simulink model "tsc_control_red"  (R2024a)
settings: Solver=ode15s  StartTime=0.0  StopTime=tm_final  MaxStep=tm_h  RelTol=1e-9  AbsTol=1e-11
model workspace (MAT data in the model file):
  tm_C1 = 1.87501784269e-05
  tm_C2 = 3.75003568539e-05
  tm_Cp = 2.89288467158e-06
  tm_L1 = 0.26018031666
  tm_L2 = 0.13009015833
  tm_Lg = 0.0008
  tm_R1 = 1.15690788571
  tm_R2 = 0.578453942857
  tm_Rb1 = 84640
  tm_Rb2 = 42320
  tm_Rg = 0.4
  tm_Rp = 2.20064
  tm_a1 = 1
  tm_a2 = 0.03
  tm_a3 = 0.03
  tm_carga = [0 1e-05 2e-05 3e-05 4e-05 5e-05 6e-05 7e-05 8e-05 9e-05 0.0001 0.00011 ... (160002 elements, 80001x2)]
  tm_final = 0.8
  tm_h = 2.5e-05
  tm_iG0 = 2.93102214056
  tm_lambda = 229.793279031
  tm_omega = 314.159265359
  tm_vC10 = 0
  tm_vC20 = 0
  tm_vCp0 = 342.613901809
  tsc_cfg.p.L_H = [0.26018031666 0.13009015833]
  tsc_cfg.p.C_F = [1.87501784269e-05 3.75003568539e-05]
  tsc_cfg.p.R_ohm = [1.15690788571 0.578453942857]
  tsc_cfg.p.Rb_ohm = [84640 42320]
  tsc_cfg.p.Cp_F = 2.89288467158e-06
  tsc_cfg.p.Rp_ohm = 2.20064
  tsc_cfg.p.omega = 314.159265359
  tsc_cfg.p.T = 0.02
  tsc_cfg.p.lambda = 229.793279031
  tsc_cfg.p.k = 42.32
  tsc_cfg.p.coefTension = [1 0.03 0.03]
  tsc_cfg.p.limiteDiDt_A_s = 2500
  tsc_cfg.p.limiteDiDtPlan_A_s = 2475
  tsc_cfg.p.margenDiDt = 0.01
  tsc_cfg.p.permanenciaMin_s = 0.06
  tsc_cfg.p.histeresis_A2 = 0.025
  tsc_cfg.p.pasoMuestreo_s = 0.00031746031746
  tsc_cfg.p.ruidoSigma_A = 0
  tsc_cfg.p.PNominal_W = 1000
  tsc_cfg.p.opciones.CasoTension = "moderada"
  tsc_cfg.p.opciones.Modo = "ga"
  tsc_cfg.p.opciones.BitsFijos = [1 0]
  tsc_cfg.p.opciones.PNominal_W = 1000
  tsc_cfg.p.opciones.Duracion_s = 0.8
  tsc_cfg.p.opciones.PasoMaximo_s = 2.5e-05
  tsc_cfg.p.opciones.VCInicial_V = [0 0]
  tsc_cfg.p.opciones.MaxDiDt_A_s = 2500
  tsc_cfg.p.opciones.Permanencia_s = 0.06
  tsc_cfg.p.opciones.Histeresis_A2 = 0.025
  tsc_cfg.p.opciones.MargenDiDt = 0.01
  tsc_cfg.p.opciones.EscalaCarga = [0.45 1.35 0.55 1.15]
  tsc_cfg.p.opciones.InstantesCarga_s = [0 0.2 0.4 0.6]
  tsc_cfg.p.opciones.Transicion_s = 0.06
  tsc_cfg.p.uReferencia = [344.475378053; 342.234056862; 335.572294082; 324.672808973; 309.827507389; 291.419626131; 269.900805928; 245.76494729; 219.520945261; 191.666460359; 162.664759213; 132.926361149; 102.796783137; 72.5511245888; 42.3956243918; 12.4757090319; -17.1105133821; -46.2948235646; -75.0193622969; -103.216997622; -130.793561892; -157.613734298; -183.491988067; -208.189539599; -231.417673404; -252.847222623; -272.123413738; -288.884787089; -302.784526411; -313.512304625; -320.814699368; -324.512354836; -324.512354836; -320.814699368; -313.512304625; -302.784526411; -288.884787089; -272.123413738; -252.847222623; -231.417673404; -208.189539599; -183.491988067; -157.613734298; -130.793561892; -103.216997622; -75.0193622969; -46.2948235646; -17.1105133821; 12.4757090319; 42.3956243918; 72.5511245888; 102.796783137; 132.926361149; 162.664759213; 191.666460359; 219.520945261; 245.76494729; 269.900805928; 291.419626131; 309.827507389; 324.672808973; 335.572294082; 342.234056862]
  tsc_cfg.p.iCargaReferencia = [6.51182189137; 7.16575638416; 7.73235116479; 8.21110783281; 8.60326005793; 8.91131348924; 9.13853778462; 9.2884553265; 9.3643709259; 9.36898275933; 9.30410728819; 9.17054063334; 8.96806671553; 8.69560948452; 8.35151387567; 7.9339288523; 7.44125698892; 6.87262928743; 6.22836178092; 5.51035213356; 4.72237972346; 3.87028111377; 2.9619836181; 2.00739188717; 1.01813500096; 0.00719333849221; -1.01156551506; -2.02390524428; -3.01575305312; -3.97370466865; -4.88546429102; -5.74018819674; -6.52870990668; -7.24363587413; -7.87931251943; -8.43167705693; -8.89801487251; -9.27665428601; -9.56663464748; -9.76738541319; -9.87845198541; -9.89929885692; -9.8292124672; -9.66731590084; -9.41269608903; -9.0646325672; -8.62290617078; -8.08815730582; -7.46225743332; -6.74865473042; -5.95265581387; -5.08160988616; -4.14496932337; -3.15421090963; -2.12261374764; -1.06490229599; 0.00322510035915; 1.06565147543; 2.10644175202; 3.11044532539; 4.06385658961; 4.95469208973; 5.77314935733]
  tsc_cfg.p.cpReferencia = [0.000821056838438 -0.0399433156679 -0.0796021803624 -0.11709608866 -0.151499211358 -0.182073153192 -0.208305554993 -0.229930479172 -0.246929145209 -0.259511271415 -0.268078939042 -0.273176379618 ... (126 elements, 63x2)]
  tsc_cfg.p.x0 = [0; 0; 0; 0; 0; 0]
  tsc_cfg.p.bits = [0  0; 0  1; 1  0; 1  1]
  tsc_cfg.D63 = [0 -10.0309181665 5.02170145378 -3.3547530699 2.52339001873 -2.02628170292 1.69632306201 -1.46190220008 1.28721732655 -1.15238243548 1.04546960893 -0.958891913625 ... (3969 elements, 63x63)]
  tsc_cfg.Modo = "ga"
  tsc_cfg.BitsFijos = [1 0]
  tsc_cfg.TsSupervision = 0.00031746031746
  tsc_cfg.Duracion_s = 0.8
  tsc_cfg.PasoMaximo_s = 2.5e-05
  tsc_cfg.VCInicial_V = [0 0]
  tsc_cfg.CasoTension = "moderada"
  tsc_cfg.opciones.CasoTension = "moderada"
  tsc_cfg.opciones.Modo = "ga"
  tsc_cfg.opciones.BitsFijos = [1 0]
  tsc_cfg.opciones.PNominal_W = 1000
  tsc_cfg.opciones.Duracion_s = 0.8
  tsc_cfg.opciones.PasoMaximo_s = 2.5e-05
  tsc_cfg.opciones.VCInicial_V = [0 0]
  tsc_cfg.opciones.MaxDiDt_A_s = 2500
  tsc_cfg.opciones.Permanencia_s = 0.06
  tsc_cfg.opciones.Histeresis_A2 = 0.025
  tsc_cfg.opciones.MargenDiDt = 0.01
  tsc_cfg.opciones.EscalaCarga = [0.45 1.35 0.55 1.15]
  tsc_cfg.opciones.InstantesCarga_s = [0 0.2 0.4 0.6]
  tsc_cfg.opciones.Transicion_s = 0.06
  tsc_cfg.CargaExogena = [0 1e-05 2e-05 3e-05 4e-05 5e-05 6e-05 7e-05 8e-05 9e-05 0.0001 0.00011 ... (160002 elements, 80001x2)]
  tsc_cfg.vCp0 = 342.613901809
  tsc_cfg.alcance = "Simulacion con predictor temporal de red y limites condicionales de arranque. e se mide aguas arriba; carga reconstruida localmente. Se repite el ultimo periodo, sin anticipar rampas. No garantiza limites frente a excitaciones futuras arbitrarias."
  tsc_cfg.Fuente.R_ohm = 0.4
  tsc_cfg.Fuente.L_H = 0.0008
  tsc_cfg.Fuente.i0_A = 2.93102214056
  tsc_cfg.Fuente.referenciaInicial.u = [342.615447295; 340.36933981; 333.716987001; 322.838832299; 308.024877704; 289.656978152; 268.186008364; 244.105748993; 217.925586147; 190.14418538; 161.226182754; 131.583642897; 101.563593418; 71.4423959692; 41.4271053381; 11.6633529109; -17.7512761437; -46.7498720667; -75.2766672263; -103.267335864; -130.631106571; -157.236473824; -182.901942383; -207.392759034; -230.424023811; -251.669978153; -270.778694185; -287.390888758; -301.161203003; -311.780056943; -318.994129669; -322.623633642; -322.574835789; -318.846702354; -311.531070434; -300.806329117; -286.925174715; -270.197535167; -250.970190107; -229.604906391; -206.457037157; -181.856483906; -156.092699593; -129.405035852; -101.979242671; -73.9503582505; -45.4116318061; -16.4285560767; 12.9433993556; 42.6391241117; 72.5642462132; 102.577554907; 132.477313799; 161.992989188; 190.783456274; 218.442183277; 244.509279799; 268.489684811; 289.876215396; 308.175749026; 322.936509575; 333.774297792; 340.395562704]
  tsc_cfg.Fuente.referenciaInicial.e = [344.475378053; 342.234056862; 335.572294082; 324.672808973; 309.827507389; 291.419626131; 269.900805928; 245.76494729; 219.520945261; 191.666460359; 162.664759213; 132.926361149; 102.796783137; 72.5511245888; 42.3956243918; 12.4757090319; -17.1105133821; -46.2948235646; -75.0193622969; -103.216997622; -130.793561892; -157.613734298; -183.491988067; -208.189539599; -231.417673404; -252.847222623; -272.123413738; -288.884787089; -302.784526411; -313.512304625; -320.814699368; -324.512354836; -324.512354836; -320.814699368; -313.512304625; -302.784526411; -288.884787089; -272.123413738; -252.847222623; -231.417673404; -208.189539599; -183.491988067; -157.613734298; -130.793561892; -103.216997622; -75.0193622969; -46.2948235646; -17.1105133821; 12.4757090319; 42.3956243918; 72.5511245888; 102.796783137; 132.926361149; 162.664759213; 191.666460359; 219.520945261; 245.76494729; 269.900805928; 291.419626131; 309.827507389; 324.672808973; 335.572294082; 342.234056862]
  tsc_cfg.Fuente.referenciaInicial.iFuente = [2.93102214056; 3.18466917969; 3.40009695268; 3.57814315406; 3.72029288696; 3.82841734815; 3.9045060869; 3.95041594506; 3.96765809945; 3.95724111143; 3.91958285068; 3.85449804158; 3.76126151507; 3.63874061709; 3.48558420243; 3.30045075069; 3.08225479922; 2.83040937826; 2.54504257797; 2.22716872259; 1.87879865753; 1.5029790038; 1.10375642318; 0.686069414865; 0.255576357856; -0.181566121863; -0.618956312321; -1.05021153612; -1.46922208838; -1.8703751595; -2.24873197036; -2.60014586812; -2.9213146946; -3.20976683435; -3.46378642066; -3.6822886735; -3.86466076463; -4.01058655424; -4.11987475435; -4.1923094407; -4.22753941769; -4.22501896306; -4.18400730545; -4.10362829346; -3.98298563955; -3.82132342581; -3.61821676754; -3.37377409126; -3.08883072315; -2.76511357784; -2.4053586967; -2.01336705046; -1.59398908149; -1.15303447661; -0.697110103385; -0.233395342802; 0.230630353317; 0.687488461278; 1.13000893641; 1.55162138892; 1.9466079948; 2.3102991732; 2.63919762427]
  tsc_cfg.Fuente.referenciaInicial.iCarga = [2.93031985112; 3.22459037287; 3.47955802416; 3.69499852476; 3.87146702607; 4.01009107016; 4.11234200308; 4.17980489692; 4.21396691665; 4.2160422417; 4.18684827969; 4.126743285; 4.03563002199; 3.91302426804; 3.75818124405; 3.57026798353; 3.34856564501; 3.09268317934; 2.80276280142; 2.4796584601; 2.12507087556; 1.7416265012; 1.33289262814; 0.903326349225; 0.45816075043; 0.0032370023215; -0.455204481777; -0.910757359924; -1.3570888739; -1.78816710089; -2.19845893096; -2.58308468853; -2.93791945801; -3.25963614336; -3.54569063374; -3.79425467562; -4.00410669263; -4.17449442871; -4.30498559136; -4.39532343594; -4.44530339343; -4.45468448561; -4.42314561024; -4.35029215538; -4.23571324006; -4.07908465524; -3.88030777685; -3.63967078762; -3.35801584499; -3.03689462869; -2.67869511624; -2.28672444877; -1.86523619552; -1.41939490934; -0.95517618644; -0.479206033195; 0.00145129516162; 0.479543163942; 0.947898788408; 1.39970039643; 1.82873546532; 2.22961144038; 2.5979172108]
  tsc_cfg.Fuente.referenciaInicial.iCp = [0.000702289439303; -0.0399211931839; -0.0794610714726; -0.116855370706; -0.151174139109; -0.181673722008; -0.207835916181; -0.229388951867; -0.246308817205; -0.25880113027; -0.267265429006; -0.272245243421; -0.274368506918; -0.274283650945; -0.272597041625; -0.26981723284; -0.266310845793; -0.262273801084; -0.257720223447; -0.252489737507; -0.246272218026; -0.238647497399; -0.229136204962; -0.21725693436; -0.202584392574; -0.184803124184; -0.163751830545; -0.1394541762; -0.112133214471; -0.0822080586042; -0.0502730393974; -0.017061179585; 0.0166047634053; 0.0498693090126; 0.0819042130854; 0.111966002121; 0.139445927998; 0.163907874464; 0.185110837015; 0.203013995238; 0.217763975741; 0.229665522555; 0.23913830479; 0.246663861916; 0.252727600509; 0.257761229424; 0.262091009311; 0.265896696354; 0.269185121845; 0.271781050855; 0.273336419545; 0.273357398316; 0.271247114027; 0.26636043273; 0.258066083055; 0.245810690393; 0.229179058156; 0.207945297336; 0.182110148004; 0.151920992488; 0.117872529477; 0.0806877328153; 0.0412804134728]
  tsc_cfg.Fuente.referenciaInicial.vCp = [342.613901809; 340.457191985; 333.891852214; 323.095988902; 308.357557562; 290.056776611; 268.643380394; 244.610551496; 218.467623182; 190.713713499; 161.814337748; 132.18275667; 102.167379729; 72.0459955428; 42.0269932918; 12.2571235062; -17.165221844; -46.172701849; -74.7095177938; -102.711696848; -130.089150077; -156.711296596; -182.397696085; -206.914654734; -229.978208493; -251.263293006; -270.418335357; -287.08400032; -300.914438166; -311.599146601; -318.883496807; -322.586088128; -322.611376895; -318.95644675; -311.711312122; -301.05272598; -287.232045002; -270.558237392; -251.377552419; -230.051667109; -206.936257272; -182.361895042; -156.618956912; -129.947854213; -102.535405138; -74.5175979224; -45.9883997648; -17.0136989826; 12.3510198091; 42.0410318599; 71.9627311549; 101.975993682; 131.88039655; 161.406825765; 190.215545729; 217.901242439; 244.004939196; 268.032072072; 289.47545652; 307.841425613; 322.677114572; 333.59673314; 340.304719375]
  tsc_cfg.Fuente.referenciaInicial.iRamas = [0  0; 0  0; 0  0; 0  0; 0  0; 0  0; 0  0; 0  0; 0  0; 0  0; 0  0; 0  0; 0  0; 0  0; 0  0; 0  0; 0  0; 0  0; 0  0; 0  0; 0  0; 0  0; 0  0; 0  0; 0  0; 0  0; 0  0; 0  0; 0  0; 0  0; 0  0; 0  0; 0  0; 0  0; 0  0; 0  0; 0  0; 0  0; 0  0; 0  0; 0  0; 0  0; 0  0; 0  0; 0  0; 0  0; 0  0; 0  0; 0  0; 0  0; 0  0; 0  0; 0  0; 0  0; 0  0; 0  0; 0  0; 0  0; 0  0; 0  0; 0  0; 0  0; 0  0]
  tsc_cfg.Fuente.referenciaInicial.vCs = [0  0; 0  0; 0  0; 0  0; 0  0; 0  0; 0  0; 0  0; 0  0; 0  0; 0  0; 0  0; 0  0; 0  0; 0  0; 0  0; 0  0; 0  0; 0  0; 0  0; 0  0; 0  0; 0  0; 0  0; 0  0; 0  0; 0  0; 0  0; 0  0; 0  0; 0  0; 0  0; 0  0; 0  0; 0  0; 0  0; 0  0; 0  0; 0  0; 0  0; 0  0; 0  0; 0  0; 0  0; 0  0; 0  0; 0  0; 0  0; 0  0; 0  0; 0  0; 0  0; 0  0; 0  0; 0  0; 0  0; 0  0; 0  0; 0  0; 0  0; 0  0; 0  0; 0  0]
  tsc_cfg.Fuente.referenciaInicial.I_fuente_RMS_A = 2.97261097458
  tsc_cfg.Fuente.referenciaInicial.U_RMS_V = 228.658602065
  tsc_cfg.Fuente.referenciaInicial.P_carga_W = 446.383779747
  tsc_cfg.Fuente.referenciaInicial.P_fuente_W = 450.014334866
  tsc_cfg.Fuente.referenciaInicial.P_perdidas_W = 3.63055511908
  tsc_cfg.Fuente.referenciaInicial.Residuo_KVL_V = 2.64233079861e-13
  tsc_cfg.Fuente.referenciaInicial.Residuo_KCL_A = 4.16333634234e-16
  tsc_cfg.Fuente.referenciaInicial.Balance_W = 3.5527136788e-14
  tsc_cfg.NombreModelo = "tsc_control_red"
  tsc_cfg.ControlRed.MaxVC_V = [1100 1100]
  tsc_cfg.ControlRed.MaxI_A = [8 8]
  tsc_cfg.ControlRed.ModeloCoste = "red"
  tsc_cfg.ControlRed.Margen = 0.01
  tsc_cfg.ControlRed.PasosPlan = 126
  tsc_cfg.ControlRed.MuestrasCota = 1008
  tsc_cfg.ControlRed.Z = [0.4 -2.52104470566 1.26209123166 -0.843141407922 0.6341970836 -0.50926013696 0.426332485578 -0.367416096963 0.323512999733 -0.289625295475 0.262755171438 -0.240995823314 ... (3969 elements, 63x63)]
  tsc_cfg.ControlRed.Ycp = [0.000599610844474 -0.00946639313754 0.00463913724545 -0.00307779801005 0.00230711336453 -0.00184878505374 0.0015455876038 -0.00133067018799 0.0011707819741 -0.00104752069124 0.000949878231662 -0.000870867421724 ... (3969 elements, 63x63)]
  tsc_cfg.ControlRed.Yi = {[1.53684291055e-05 0.000711384808832 0.000506457228673 0.000558951720113 0.000429303680283 0.000417345178621 0.000296064584475 0.000252902321514 0.000132346614071 7.27845302567e-05 -4.4998037505e-05 -0.000110154353221 ... (3969 elements, 63x63)], [3.07368582109e-05 0.00142276961766 0.00101291445735 0.00111790344023 0.000858607360565 0.000834690357243 0.00059212916895 0.000505804643028 0.000264693228142 0.000145569060513 -8.999607501e-05 -0.000220308706442 ... (3969 elements, 63x63)]}
  tsc_cfg.ControlRed.Yv = {[0.0155279369362 0.0235952043446 0.033823796607 0.0428833363918 0.0512378361746 0.0584163227068 0.0644470164228 0.0690934983009 0.072342545693 0.0740699610286 0.0742883332153 0.0729594445357 ... (3969 elements, 63x63)], [0.0155279369362 0.0235952043446 0.033823796607 0.0428833363918 0.0512378361746 0.0584163227068 0.0644470164228 0.0690934983009 0.072342545693 0.0740699610286 0.0742883332153 0.0729594445357 ... (3969 elements, 63x63)]}
  tsc_cfg.ControlRed.pesos = [0.0008 2.89288467158e-06 0.26018031666 1.87501784269e-05 0.13009015833 3.75003568539e-05]
  tsc_cfg.ControlRed.escala = [0.0282842712475 0.00170084822121 0.510078735746 0.00433014762184 0.360680132985 0.00612375349389]
  tsc_cfg.ControlRed.retardos = [0 0.00015873015873 0.00031746031746 0.00047619047619 0.000634920634921 0.000793650793651 0.000952380952381 0.00111111111111 0.00126984126984 0.00142857142857 0.0015873015873 0.00174603174603 ... (127 elements, 127x1)]
  tsc_cfg.ControlRed.Kplan = [1 0.636685738197 3.89978788099e-17 -0.212404603169 -3.90464165819e-17 0.127654358683 3.9127501038e-17 -0.091409055288 -3.92414159929e-17 0.0713326858323 -7.48780844669e-17 -0.0586065146832 ... (8001 elements, 127x63)]
  tsc_cfg.ControlRed.Kcota = [1 0.993588459691 0.974501668983 0.943179063132 0.900339637331 0.846962271352 0.784259010486 0.713642098008 0.636685738197 0.555083722074 0.470604165854 0.385042690993 ... (63504 elements, 1008x63)]
  tsc_cfg.ControlRed.topologias{1}.Ue = [1.08699749191 -0.0484972288162 0.0114250159703 -0.00380936220767 0.00130822478792 -0.000275246456701 -0.000210343928743 0.000456400434896 -0.000585894193282 0.000654367272004 -0.000689253987996 0.000705050503954 ... (3969 elements, 63x63)]
  tsc_cfg.ControlRed.topologias{1}.Ul = [-0.507868422778 2.84703126305 -1.57599831145 1.07560773838 -0.81464964244 0.655922159162 -0.549734587263 0.473987684451 -0.417416712339 0.373694352289 -0.338999159098 0.310889604765 ... (3969 elements, 63x63)]
  tsc_cfg.ControlRed.topologias{1}.Y = [0.000599610844474 -0.00946639313754 0.00463913724545 -0.00307779801005 0.00230711336453 -0.00184878505374 0.0015455876038 -0.00133067018799 0.0011707819741 -0.00104752069124 0.000949878231662 -0.000870867421724 ... (3969 elements, 63x63)]
  tsc_cfg.ControlRed.topologias{1}.A = [-3250.8  -1250  2750.8  0  2750.8  0; 345675.72286  0  -345675.72286  0  -345675.72286  0; 0  0  0  0  0  0; 0  0  0  -0.63011372652  0  0; 0  0  0  0  0  0; 0  0  0  0  0  -0.63011372652]
  tsc_cfg.ControlRed.topologias{1}.F = [1 0 0 0 0 0 0 1 0 0 0 0 ... (4572 elements, 6x6x127)]
  tsc_cfg.ControlRed.topologias{2}.Ue = [1.07982847686 -0.0483136101854 0.0110994946165 -0.00394544501447 0.00128605797666 -0.000247931808284 -2.69704122161e-05 0.000671993779742 -0.000221335812626 0.00104141425263 -0.000173221739429 0.00122927774362 ... (3969 elements, 63x63)]
  tsc_cfg.ControlRed.topologias{2}.Ul = [-0.501129099659 2.82693894373 -1.56412785791 1.06705522919 -0.808503052804 0.650505569149 -0.545718937968 0.469935677557 -0.414486155118 0.370398933376 -0.336703532122 0.308086125688 ... (3969 elements, 63x63)]
  tsc_cfg.ControlRed.topologias{2}.Y = [0.000630347702685 -0.00804362351988 0.00565205170279 -0.00195989456983 0.0031657207251 -0.0010140946965 0.00213771677275 -0.000824865544967 0.00143547520224 -0.000901951630727 0.000859882156652 -0.00109117612817 ... (3969 elements, 63x63)]
  tsc_cfg.ControlRed.topologias{2}.A = [-3250.8  -1250  2750.8  0  2750.8  0; 345675.72286  0  -345675.72286  0  -345675.72286  0; 0  0  0  0  0  0; 0  0  0  -0.63011372652  0  0; 16.9162681347  7.68697657714  -16.9162681347  0  -21.3628300444  -7.68697657714; 0  0  0  0  26666.4129063  -0.63011372652]
  tsc_cfg.ControlRed.topologias{2}.F = [1 0 0 0 0 0 0 1 0 0 0 0 ... (4572 elements, 6x6x127)]
  tsc_cfg.ControlRed.topologias{3}.Ue = [1.08340123426 -0.0484056938576 0.0112604388549 -0.00387930449402 0.00129525724348 -0.00026375902484 -0.000120593732726 0.000562085886112 -0.000405389163691 0.00084606476122 -0.00043265941419 0.000965783588098 ... (3969 elements, 63x63)]
  tsc_cfg.ControlRed.topologias{3}.Ul = [-0.5044804513 2.8369506267 -1.57003889598 1.07131636046 -0.811562812992 0.653204667116 -0.547717534046 0.471954949682 -0.415944593241 0.372041112417 -0.337846070667 0.309482976505 ... (3969 elements, 63x63)]
  tsc_cfg.ControlRed.topologias{3}.Y = [0.00061497927358 -0.00875500832871 0.00514559447412 -0.00251884628994 0.00273641704482 -0.00143143987512 0.00184165218827 -0.00107776786648 0.00130312858817 -0.000974736160983 0.000904880194157 -0.000981021774945 ... (3969 elements, 63x63)]
  tsc_cfg.ControlRed.topologias{3}.A = [-3250.8  -1250  2750.8  0  2750.8  0; 345675.72286  0  -345675.72286  0  -345675.72286  0; 8.45813406736  3.84348828857  -12.9046959771  -3.84348828857  -8.45813406736  0; 0  0  53332.8258127  -0.63011372652  0  0; 0  0  0  0  0  0; 0  0  0  0  0  -0.63011372652]
  tsc_cfg.ControlRed.topologias{3}.F = [1 0 0 0 0 0 0 1 0 0 0 0 ... (4572 elements, 6x6x127)]
  tsc_cfg.ControlRed.topologias{4}.Ue = [1.0762790017 -0.0482209852552 0.010942127268 -0.00400785634311 0.0012805458148 -0.000227866259732 7.04237550423e-05 0.000786008012448 -3.38447531466e-05 0.00124029928139 8.89544368334e-05 0.00149543024097 ... (3969 elements, 63x63)]
  tsc_cfg.ControlRed.topologias{4}.Ul = [-0.497813857674 2.81699550499 -1.55826460896 1.06282403687 -0.805470003092 0.647824695936 -0.543738540098 0.467929752754 -0.413041201477 0.368767718317 -0.33557139594 0.30669895587 ... (3969 elements, 63x63)]
  tsc_cfg.ControlRed.topologias{4}.Y = [0.000645716131791 -0.00733223871105 0.00615850893147 -0.00140094284971 0.00359502440538 -0.000596749517875 0.00243378135722 -0.000571963223453 0.00156782181631 -0.00082916710047 0.000814884119147 -0.00120133048139 ... (3969 elements, 63x63)]
  tsc_cfg.ControlRed.topologias{4}.A = [-3250.8  -1250  2750.8  0  2750.8  0; 345675.72286  0  -345675.72286  0  -345675.72286  0; 8.45813406736  3.84348828857  -12.9046959771  -3.84348828857  -8.45813406736  0; 0  0  53332.8258127  -0.63011372652  0  0; 16.9162681347  7.68697657714  -16.9162681347  0  -21.3628300444  -7.68697657714; 0  0  0  0  26666.4129063  -0.63011372652]
  tsc_cfg.ControlRed.topologias{4}.F = [1 0 0 0 0 0 0 1 0 0 0 0 ... (4572 elements, 6x6x127)]
(part 1 of 2)
Description:
  | Simulacion con predictor temporal de red y limites condicionales de arranque. e se mide aguas arriba; carga reconstruida localmente. Se repite el ultimo periodo, sin anticipar rampas. No garantiza limites frente a excitaciones futuras arbitrarias.
settings Model: Creator=paco  LastModifiedBy=paco
settings DataIOCC: SaveOutput=off  SignalLogging=off  SaveTime=off
settings DebuggingCC: AlgebraicLoopMsg=error

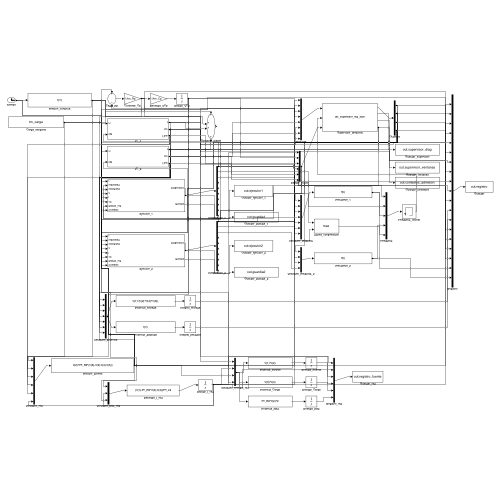
[thumbnail: Simulink's stored preview of the top-level diagram]
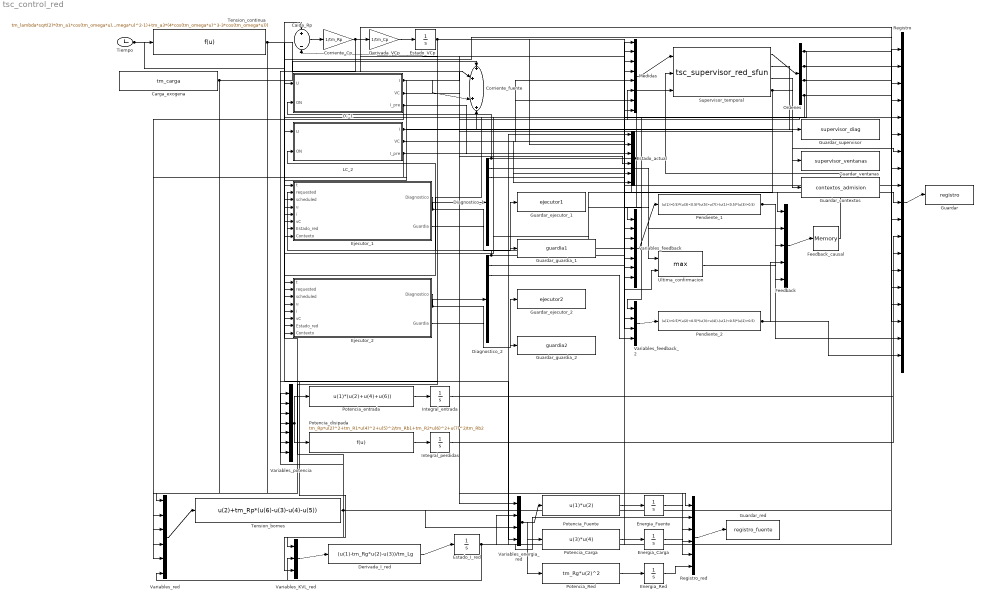
== system tsc_control_red ==
  Caida_Rp : Sum  Inputs=+-
  Carga_exogena : FromWorkspace  VariableName=tm_carga  OutputAfterFinalValue=Holding final value
  Corriente_Cp : Gain  Gain=1/tm_Rp
  Corriente_fuente : Sum  Inputs=++++
  Derivada_I_red : Fcn  Expr=(u(1)-tm_Rg*u(2)-u(3))/tm_Lg
  Derivada_VCp : Gain  Gain=1/tm_Cp
  Diagnostico_1 : Demux  Outputs=10
  Diagnostico_2 : Demux  Outputs=10
  Ejecutor_1 : Subsystem
  Ejecutor_2 : Subsystem
  Energia_Carga : Integrator
  Energia_Fuente : Integrator
  Energia_Red : Integrator
  Estado_I_red : Integrator  InitialCondition=tm_iG0
  Estado_VCp : Integrator  InitialCondition=tm_vCp0
  Estado_actual : Mux  Inputs=6
  Feedback : Mux  Inputs=5
  Feedback_causal : Memory  InitialCondition=[0;0;0;0;-1e6]
  Guardar : ToWorkspace  VariableName=registro  SaveFormat=Timeseries  SampleTime=-1
  Guardar_contextos : ToWorkspace  VariableName=contextos_admision  SaveFormat=Timeseries  SampleTime=tsc_cfg.p.T
  Guardar_ejecutor_1 : ToWorkspace  VariableName=ejecutor1  SaveFormat=Timeseries  SampleTime=-1
  Guardar_ejecutor_2 : ToWorkspace  VariableName=ejecutor2  SaveFormat=Timeseries  SampleTime=-1
  Guardar_guardia_1 : ToWorkspace  VariableName=guardia1  SaveFormat=Timeseries  SampleTime=tsc_cfg.TsSupervision
  Guardar_guardia_2 : ToWorkspace  VariableName=guardia2  SaveFormat=Timeseries  SampleTime=tsc_cfg.TsSupervision
  Guardar_red : ToWorkspace  VariableName=registro_fuente  SaveFormat=Timeseries  SampleTime=-1
  Guardar_supervisor : ToWorkspace  VariableName=supervisor_diag  SaveFormat=Timeseries  SampleTime=tsc_cfg.TsSupervision
  Guardar_ventanas : ToWorkspace  VariableName=supervisor_ventanas  SaveFormat=Timeseries  SampleTime=tsc_cfg.p.T
  Integral_entrada : Integrator
  Integral_perdidas : Integrator
  LC_1 : Subsystem
  LC_2 : Subsystem
  Medidas : Mux  Inputs=8
  Ordenes : Demux
  Pendiente_1 : Fcn  Expr=(u(1)>0.5)*(u(3)<0.5)*(u(5)>u(7))-(u(1)<0.5)*(u(3)>0.5)
  Pendiente_2 : Fcn  Expr=(u(1)>0.5)*(u(2)<0.5)*(u(3)>u(4))-(u(1)<0.5)*(u(2)>0.5)
  Potencia_Carga : Fcn  Expr=u(3)*u(4)
  Potencia_Fuente : Fcn  Expr=u(1)*u(2)
  Potencia_Red : Fcn  Expr=tm_Rg*u(2)^2
  Potencia_disipada : Fcn  Expr=tm_Rp*u(2)^2+tm_R1*u(4)^2+u(5)^2/tm_Rb1+tm_R2*u(6)^2+u(7)^2/tm_Rb2
  Potencia_entrada : Fcn  Expr=u(1)*(u(2)+u(4)+u(6))
  Registro : Mux  Inputs=19
  Registro_red : Mux  Inputs=6
  Supervisor_temporal : M-S-Function  FunctionName=tsc_supervisor_red_sfun  Parameters=tsc_cfg
  Tension_bornes : Fcn  Expr=u(2)+tm_Rp*(u(6)-u(3)-u(4)-u(5))
  Tension_continua : Fcn  Expr=tm_lambda*sqrt(2)*(tm_a1*cos(tm_omega*u)+tm_a2*(2*cos(tm_omega*u)^2-1)+tm_a3*(4*cos(tm_omega*u)^3-3*cos(tm_omega*u)))
  Tiempo : Clock
  Ultima_confirmacion : MinMax  Function=max  Inputs=2
  Variables_KVL_red : Mux  Inputs=3
  Variables_energia_red : Mux
  Variables_feedback : Mux  Inputs=7
  Variables_feedback_2 : Mux
  Variables_potencia : Mux  Inputs=7
  Variables_red : Mux  Inputs=6
  wires:
  Tiempo/1 -> Tension_continua/1, Ejecutor_1/1(t), Ejecutor_2/1(t)
  Estado_VCp/1 -> Caida_Rp/2, Variables_potencia/3, Registro/5, Variables_red/2, Estado_actual/2
  Caida_Rp/1 -> Corriente_Cp/1
  Corriente_Cp/1 -> Derivada_VCp/1, Corriente_fuente/2, Medidas/3, Variables_potencia/2, Registro/4
  Derivada_VCp/1 -> Estado_VCp/1
  Carga_exogena/1 -> Corriente_fuente/1, Registro/2, Variables_red/3, Variables_energia_red/4
  Diagnostico_1/1 -> LC_1/2(ON), Variables_feedback/3, Feedback/1, Registro/10
  LC_1/1(I) -> Corriente_fuente/3, Medidas/4, Variables_potencia/4, Registro/6
  Ordenes/1 -> Ejecutor_1/2(requested), Variables_feedback/1, Registro/14
  Ordenes/3 -> Ejecutor_1/3(scheduled), Variables_feedback/5, Registro/16
  LC_1/3(I_pre) -> Ejecutor_1/5(i), Variables_red/4, Estado_actual/3
  LC_1/2(VC) -> Ejecutor_1/6(vC), Medidas/6, Variables_potencia/5, Registro/7, Estado_actual/4
  Ejecutor_1/1(Diagnostico) -> Diagnostico_1/1, Guardar_ejecutor_1/1
  Diagnostico_2/1 -> LC_2/2(ON), Variables_feedback/4, Variables_feedback_2/2, Feedback/2, Registro/11
  LC_2/1(I) -> Corriente_fuente/4, Medidas/5, Variables_potencia/6, Registro/8
  Ordenes/2 -> Ejecutor_2/2(requested), Variables_feedback/2, Variables_feedback_2/1, Registro/15
  Ordenes/4 -> Ejecutor_2/3(scheduled), Variables_feedback/6, Variables_feedback_2/3, Registro/17
  LC_2/3(I_pre) -> Ejecutor_2/5(i), Variables_red/5, Estado_actual/5
  LC_2/2(VC) -> Ejecutor_2/6(vC), Medidas/7, Variables_potencia/7, Registro/9, Estado_actual/6
  Ejecutor_2/1(Diagnostico) -> Diagnostico_2/1, Guardar_ejecutor_2/1
  Medidas/1 -> Supervisor_temporal/1
  Feedback_causal/1 -> Supervisor_temporal/2
  Supervisor_temporal/1 -> Ordenes/1
  Supervisor_temporal/2 -> Guardar_supervisor/1
  Supervisor_temporal/3 -> Guardar_ventanas/1
  Diagnostico_1/3 -> Variables_feedback/7
  Diagnostico_2/3 -> Variables_feedback_2/4
  Variables_feedback/1 -> Pendiente_1/1
  Variables_feedback_2/1 -> Pendiente_2/1
  Diagnostico_1/2 -> Ultima_confirmacion/1
  Diagnostico_2/2 -> Ultima_confirmacion/2
  Pendiente_1/1 -> Feedback/3, Registro/18
  Pendiente_2/1 -> Feedback/4, Registro/19
  Ultima_confirmacion/1 -> Feedback/5
  Feedback/1 -> Feedback_causal/1
  Variables_potencia/1 -> Potencia_entrada/1, Potencia_disipada/1
  Potencia_entrada/1 -> Integral_entrada/1
  Potencia_disipada/1 -> Integral_perdidas/1
  Integral_entrada/1 -> Registro/12
  Integral_perdidas/1 -> Registro/13
  Registro/1 -> Guardar/1
  Tension_continua/1 -> Variables_KVL_red/1, Variables_red/1, Variables_energia_red/1, Registro_red/1, Medidas/8
  Estado_I_red/1 -> Variables_KVL_red/2, Variables_red/6, Medidas/2, Registro/3, Variables_energia_red/2, Registro_red/2, Estado_actual/1
  Tension_bornes/1 -> Variables_KVL_red/3, Caida_Rp/1, LC_1/1(U), Ejecutor_1/4(u), LC_2/1(U), Ejecutor_2/4(u), Medidas/1, Variables_potencia/1, Registro/1, Variables_energia_red/3, Registro_red/3
  Variables_KVL_red/1 -> Derivada_I_red/1
  Derivada_I_red/1 -> Estado_I_red/1
  Variables_red/1 -> Tension_bornes/1
  Variables_energia_red/1 -> Potencia_Fuente/1, Potencia_Carga/1, Potencia_Red/1
  Potencia_Fuente/1 -> Energia_Fuente/1
  Potencia_Carga/1 -> Energia_Carga/1
  Potencia_Red/1 -> Energia_Red/1
  Energia_Fuente/1 -> Registro_red/4
  Energia_Carga/1 -> Registro_red/5
  Energia_Red/1 -> Registro_red/6
  Registro_red/1 -> Guardar_red/1
  Estado_actual/1 -> Supervisor_temporal/3, Ejecutor_1/7(Estado_red), Ejecutor_2/7(Estado_red)
  Supervisor_temporal/4 -> Guardar_contextos/1, Ejecutor_1/8(Contexto), Ejecutor_2/8(Contexto)
  Ejecutor_1/2(Guardia) -> Guardar_guardia_1/1
  Ejecutor_2/2(Guardia) -> Guardar_guardia_2/1
